simulink model "gm_comm8qamtxrxhdl"  (R2025b)
settings: Solver=FixedStepDiscrete  StartTime=0.0  StopTime=20000*qam_params.symbolPeriod  RelTol=1e-3
PreLoadFcn:
  | qam_params = comm8qamtxrxhdl_init;
InitFcn:
  | qam_params = comm8qamtxrxhdl_init;
undefined symbols (not defined in the file or in its folder): Add, Shift
libraries: simulink x4, hdlsllib x4, dspsigops x2, commchan3 x1, commrflib2 x1, dsphdlmathfun2 x1, dsphdlsigops2 x1, dspmlti4 x1, simulink_need_slupdate x1, hdlmdlgenlib x1, commdigbbndam3 x1, commsequence2 x1
(part 1 of 3)
settings Model: Creator=The MathWorks, Inc.  LastModifiedBy=Ubaid
settings SolverCC: AlgebraicLoopSolver=TrustRegion  MaxZcPerStep=1.0
settings DataIOCC: LimitDataPoints=on  SaveFormat=Array  SaveOutput=off  SaveTime=off  ReturnWorkspaceOutputs=off
settings OptimizationCC: BlockReduction=off  ConditionallyExecuteInputs=off  DefaultParameterBehavior=Inlined  ReuseModelBlockBuffer=off  LifeSpan=inf
settings DebuggingCC: AlgebraicLoopMsg=error  UnderspecifiedInitializationDetection=Classic  MergeDetectMultiDrivingBlocksExec=none  SolverPrmCheckMsg=warning  InheritedTsInSrcMsg=none  MultiTaskDSMMsg=warning  MultiTaskCondExecSysMsg=none  SingleTaskRateTransMsg=error  IntegerOverflowMsg=none  ParameterPrecisionLossMsg=none  UnconnectedInputMsg=warning  UnconnectedOutputMsg=warning  UnconnectedLineMsg=warning  AllowSymbolicDim=off  StateNameClashWarn=warning  SFUnexpectedBacktrackingDiag=warning  SFNoUnconditionalDefaultTransitionDiag=warning  SFExecutionAtInitializationDiag=none  IntegerSaturationMsg=none  ArithmeticOperatorsInVariantConditions=warning
settings HardwareCC: ProdBitPerPointer=32.0  ProdBitPerSizeT=32.0  ProdBitPerPtrDiffT=32.0  ProdLargestAtomicFloat=None  ProdIntDivRoundTo=Undefined  ProdEndianess=Unspecified  ProdWordSize=32.0  ProdHWDeviceType=ASIC/FPGA->ASIC/FPGA  ProdEqTarget=off
settings ModelReferenceCC: EnableRefExpFcnMdlSchedulingChecks=on  PropagateSignalLabelsOutOfModel=off
settings SFSimCC: SimUseLocalCustomCode=off  CustomCodeUndefinedFunction=UseInterfaceOnly
settings RTWCC: RTWUseLocalCustomCode=off  GPUComputeCapability=3.5  DLArmComputeVersion=19.05
settings CodeAppCC: StateflowObjectComments=on
settings GRTTargetCC: TargetLangStandard=C89/C90 (ANSI)
settings ConfigComp: CovMetricSettings=dw  CovSaveCumulativeToWorkspaceVar=on  CovSaveSingleToWorkspaceVar=on  CovExternalEMLEnable=off  CovSFcnEnable=off

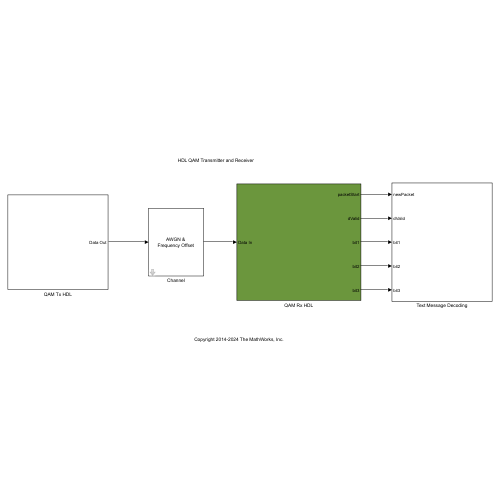
[thumbnail: Simulink's stored preview of the top-level diagram]
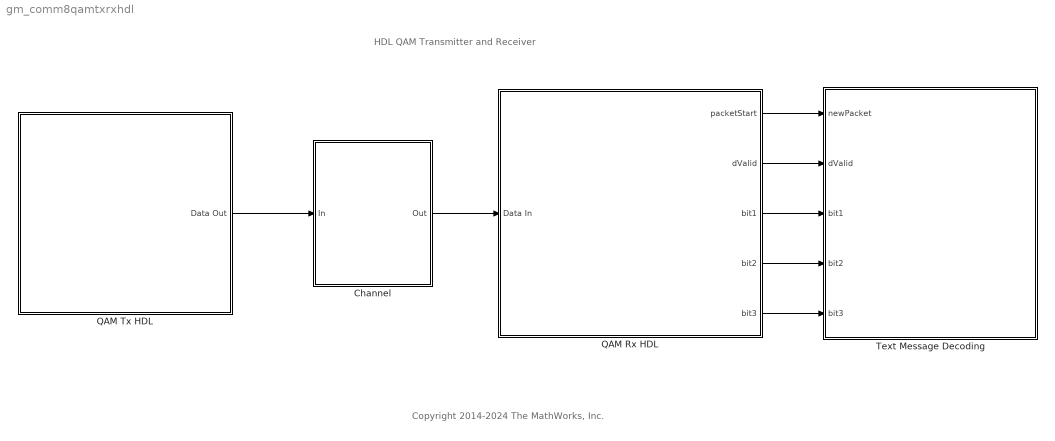
== system gm_comm8qamtxrxhdl ==
  note: HDL QAM Transmitter and Receiver
  note: Copyright 2014-2024 The MathWorks, Inc.
  Channel : Subsystem  mask{Poff=qam_params.phaseOffset, Foff=qam_params.frequencyOffset, EbNo=qam_params.EbNo, Chan_Gain=qam_params.channelGain, Chan_Delay=qam_params.channelDelay}
      mask prompts: Poff "Phase offset (deg)"; Foff "Frequency offset (Hz)"; EbNo "Eb/No"; Chan_Gain "Channel Gain"; Chan_Delay "Channel Delay"
      mask Display: disp('AWGN &\nFrequency Offset');
  QAM Rx HDL : Subsystem
  QAM Tx HDL : Subsystem
  Text Message Decoding : Subsystem
  wires:
  QAM Tx HDL/1(Data Out) -> Channel/1(In)
  Channel/1(Out) -> QAM Rx HDL/1(Data In)
  QAM Rx HDL/2(dValid) -> Text Message Decoding/2(dValid)
  QAM Rx HDL/5(bit3) -> Text Message Decoding/5(bit3)
  QAM Rx HDL/4(bit2) -> Text Message Decoding/4(bit2)
  QAM Rx HDL/3(bit1) -> Text Message Decoding/3(bit1)
  QAM Rx HDL/1(packetStart) -> Text Message Decoding/1(newPacket)

== system gm_comm8qamtxrxhdl/Channel ==
  In : Inport
  AWGN Channel2 : commchan3/AWGN Channel  LegacyMode=on  NoiseMethod="Signal to noise ratio  (Eb/No)"  noiseMode="Signal to noise ratio  (SNR)"  EbNo=EbNo  EsNo=15  SNR=15  BitsPerSymbol=3  SignalPower=0.11  SpecifySymbolPeriod=off  SamplesPerSymbol=1  SymbolPeriod=1/qam_params.sampleRate  VarianceSource=Parameter  Variance=1  RandomStream=Global stream  Seed=67  SimulateUsing=Code generation
  Constant : Constant  Value=Chan_Delay  SampleTime=1/qam_params.sampleRate
  Data Type Conversion1 : DataTypeConversion  OutDataTypeStr=fixdt(1,16,15)  SaturateOnIntegerOverflow=off  RndMeth=Floor
  Data Type Conversion4 : DataTypeConversion  OutDataTypeStr=double  SaturateOnIntegerOverflow=off  RndMeth=Floor
  Gain : Gain  Gain=Chan_Gain
  Phase/ Frequency Offset1 : commrflib2/Phase// Frequency Offset  phaseOffset=Poff  freqPort=off  freqOffset=Foff
  Variable Fractional Delay : dspsigops/Variable Fractional Delay  mode=OBSOLETE  modeActive=Linear  L=4  FarrowL=4  R=10  alpha=1  dmax=56*4  ic=0  noDFT=off  fallbackFIR=Clip to the minimum value necessary for centered kernel  fallbackFarrow=Clip to the minimum value necessary for centered kernel  roundingMode=Zero  overflowMode=off
  Out : Outport  VectorParamsAs1DForOutWhenUnconnected=off
  wires:
  Gain/1 -> Data Type Conversion1/1
  Constant/1 -> Variable Fractional Delay/2
  Variable Fractional Delay/1 -> AWGN Channel2/1
  Phase/ Frequency Offset1/1 -> Variable Fractional Delay/1
  Data Type Conversion4/1 -> Phase/ Frequency Offset1/1
  Data Type Conversion1/1 -> Out/1
  AWGN Channel2/1 -> Gain/1
  In/1 -> Data Type Conversion4/1

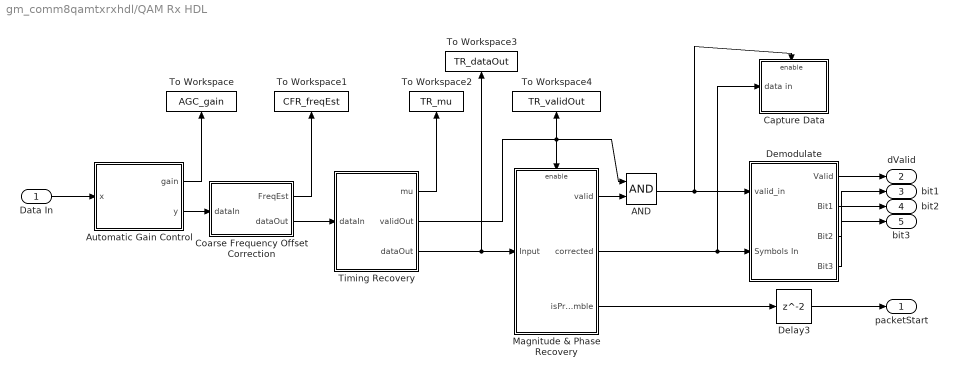
== system gm_comm8qamtxrxhdl/QAM Rx HDL ==
  Data In : Inport
  AND : Logic  AllPortsSameDT=off  OutDataTypeStr=boolean
  Automatic Gain Control : Subsystem  mask{AGC_Ref=.23, AGC_Gain=0.001}
      mask prompts: AGC_Ref "Target Amplitude"; AGC_Gain "AGC Loop Gain"
  Capture Data : Subsystem
  Coarse Frequency Offset Correction : Subsystem
  Delay3 : Delay  InitialCondition=0
  Demodulate : Subsystem
  Magnitude & Phase Recovery : Subsystem  mask{PreAmb=qam_params.preambleRx.', threshold=1.1, LMS_Step=1/4}
      mask prompts: PreAmb "Preamble symbols"; LMS_Step "LMS step size"
  Timing Recovery : Subsystem
  To Workspace : ToWorkspace  VariableName=AGC_gain  SaveFormat=Timeseries  SampleTime=-1
  To Workspace1 : ToWorkspace  VariableName=CFR_freqEst  SaveFormat=Timeseries  SampleTime=-1
  To Workspace2 : ToWorkspace  VariableName=TR_mu  SaveFormat=Timeseries  SampleTime=-1
  To Workspace3 : ToWorkspace  VariableName=TR_dataOut  SaveFormat=Timeseries  SampleTime=-1
  To Workspace4 : ToWorkspace  VariableName=TR_validOut  SaveFormat=Timeseries  SampleTime=-1
  packetStart : Outport  VectorParamsAs1DForOutWhenUnconnected=off
  dValid : Outport  Port=2  VectorParamsAs1DForOutWhenUnconnected=off
  bit1 : Outport  Port=3  VectorParamsAs1DForOutWhenUnconnected=off
  bit2 : Outport  Port=4  VectorParamsAs1DForOutWhenUnconnected=off
  bit3 : Outport  Port=5  VectorParamsAs1DForOutWhenUnconnected=off
  wires:
  Timing Recovery/1(mu) -> To Workspace2/1
  Coarse Frequency Offset Correction/1(FreqEst) -> To Workspace1/1
  Magnitude & Phase Recovery/2(corrected) -> Capture Data/1(data in), Demodulate/2(Symbols In)
  AND/1 -> Capture Data/Enable, Demodulate/1(valid_in)
  Magnitude & Phase Recovery/1(valid) -> AND/2
  Delay3/1 -> packetStart/1
  Coarse Frequency Offset Correction/2(dataOut) -> Timing Recovery/1(dataIn)
  Automatic Gain Control/2(y) -> Coarse Frequency Offset Correction/1(dataIn)
  Automatic Gain Control/1(gain) -> To Workspace/1
  Data In/1 -> Automatic Gain Control/1(x)
  Timing Recovery/2(validOut) -> Magnitude & Phase Recovery/Enable, To Workspace4/1, AND/1
  Demodulate/1(Valid) -> dValid/1
  Magnitude & Phase Recovery/3(isPreamble) -> Delay3/1
  Demodulate/4(Bit3) -> bit3/1
  Demodulate/3(Bit2) -> bit2/1
  Demodulate/2(Bit1) -> bit1/1
  Timing Recovery/3(dataOut) -> To Workspace3/1, Magnitude & Phase Recovery/1(Input)

== system gm_comm8qamtxrxhdl/QAM Tx HDL ==
  " Zero" : Constant  Value="fi(0,1,16,15,\"hex\",\"0000 + 0000 i\")"  OutDataTypeStr=fixdt(1, 16, 15)  SampleTime=1e-06
  Data Generation & Packetization : Subsystem
  Input Mux : MultiPortSwitch  DataPortOrder=Zero-based contiguous  Inputs=2  DiagnosticForDefault=None  zeroidx=on  OutDataTypeStr=fixdt(1, 16, 15)  SampleTime=1e-06  SaturateOnIntegerOverflow=off  InputSameDT=off
  Pipeline{1..4} (4 alike) : Delay  DelayLength=double(1)  InitialCondition=0  SampleTime=1e-06
  Pipeline5 : RateTransition  InitialCondition=double(0)  OutPortSampleTimeOpt=Multiple of input port sample time  OutPortSampleTimeMultiple=3
  Pipeline5_absorbed : Delay  DelayLength=0
  Pulse Shaping : Subsystem
  Symbol Mapping : Subsystem
  crp_out_delay : Delay  DelayLength=double(1)  InitialCondition=0  SampleTime=8.33333333333333e-08
  Data Out : Outport  SampleTime=2.5e-07  VectorParamsAs1DForOutWhenUnconnected=off
  wires:
  Data Generation & Packetization/1(Valid Out) -> Pipeline1/1
  Data Generation & Packetization/2(Raw Data) -> Pipeline2/1
  Symbol Mapping/1(Valid out) -> Pipeline3/1
  Pipeline1/1 -> Symbol Mapping/1(Valid In)
  Symbol Mapping/2(Symbol Out) -> Pipeline4/1
  Pipeline2/1 -> Symbol Mapping/2(Integer In)
  Pipeline3/1 -> Input Mux/1
  " Zero"/1 -> Input Mux/2
  Pipeline4/1 -> Input Mux/3
  Input Mux/1 -> Pulse Shaping/1(dataIn)
  Pulse Shaping/1(dataOut) -> crp_out_delay/1
  crp_out_delay/1 -> Pipeline5/1
  Pipeline5/1 -> Pipeline5_absorbed/1
  Pipeline5_absorbed/1 -> Data Out/1

== system gm_comm8qamtxrxhdl/Text Message Decoding ==
  newPacket : Inport
  dValid : Inport  Port=2
  bit1 : Inport  Port=3
  bit2 : Inport  Port=4
  bit3 : Inport  Port=5
  " " : MATLAB Function  TreatAsAtomicUnit=on
  Descramble and Print : Subsystem  TreatAsAtomicUnit=on
  wires:
  newPacket/1 -> " "/1(newPacket)
  dValid/1 -> " "/2(dValid)
  bit3/1 -> " "/5(bit3)
  " "/1(RxGo) -> Descramble and Print/Enable
  " "/2(framed_data) -> Descramble and Print/1(In1)
  bit2/1 -> " "/4(bit2)
  bit1/1 -> " "/3(bit1)

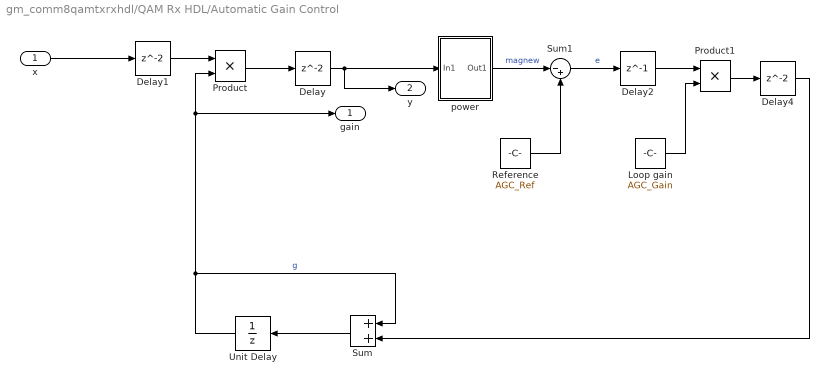
== system gm_comm8qamtxrxhdl/QAM Rx HDL/Automatic Gain Control ==
  x : Inport
  Delay : Delay  InitialCondition=0
  Delay1 : Delay  InitialCondition=0
  Delay2 : Delay  DelayLength=1  InitialCondition=0
  Delay4 : Delay  InitialCondition=0
  Loop gain : Constant  Value=AGC_Gain  OutDataTypeStr=fixdt(1,16,15)  SampleTime=1/qam_params.sampleRate
  Product : Product  OutDataTypeStr=fixdt(1,16,15)  SaturateOnIntegerOverflow=on
  Product1 : Product  OutDataTypeStr=fixdt(1,16,15)  SaturateOnIntegerOverflow=on
  Reference : Constant  Value=AGC_Ref  OutDataTypeStr=fixdt(1,16,15)  SampleTime=1/qam_params.sampleRate
  Sum : Sum  OutDataTypeStr=Inherit: Same as accumulator  AccumDataTypeStr=fixdt(1,24,15)  SaturateOnIntegerOverflow=on
  Sum1 : Sum  Inputs=|-+  OutDataTypeStr=Inherit: Same as first input
  Unit Delay : UnitDelay  InitialCondition=.5  SampleTime=-1  HasFrameUpgradeWarning=on
  power : Subsystem
  gain : Outport  VectorParamsAs1DForOutWhenUnconnected=off
  y : Outport  Port=2  PortDimensions=1  VectorParamsAs1DForOutWhenUnconnected=off
  wires:
  Delay1/1 -> Product/1
  power/1(Out1) -> Sum1/1  "magnew"
  Reference/1 -> Sum1/2
  Sum/1 -> Unit Delay/1
  Loop gain/1 -> Product1/2
  x/1 -> Delay1/1
  Delay4/1 -> Sum/2
  Unit Delay/1 -> Sum/1, Product/2, gain/1  "g"
  Product1/1 -> Delay4/1
  Delay2/1 -> Product1/1
  Sum1/1 -> Delay2/1  "e"
  Delay/1 -> power/1(In1), y/1
  Product/1 -> Delay/1

== system gm_comm8qamtxrxhdl/QAM Rx HDL/Capture Data ==
  data in : Inport
  Enable : EnablePort
  To Workspace2 : ToWorkspace  VariableName=symbolEstimates  SaveFormat=Timeseries  SampleTime=-1
  wires:
  data in/1 -> To Workspace2/1

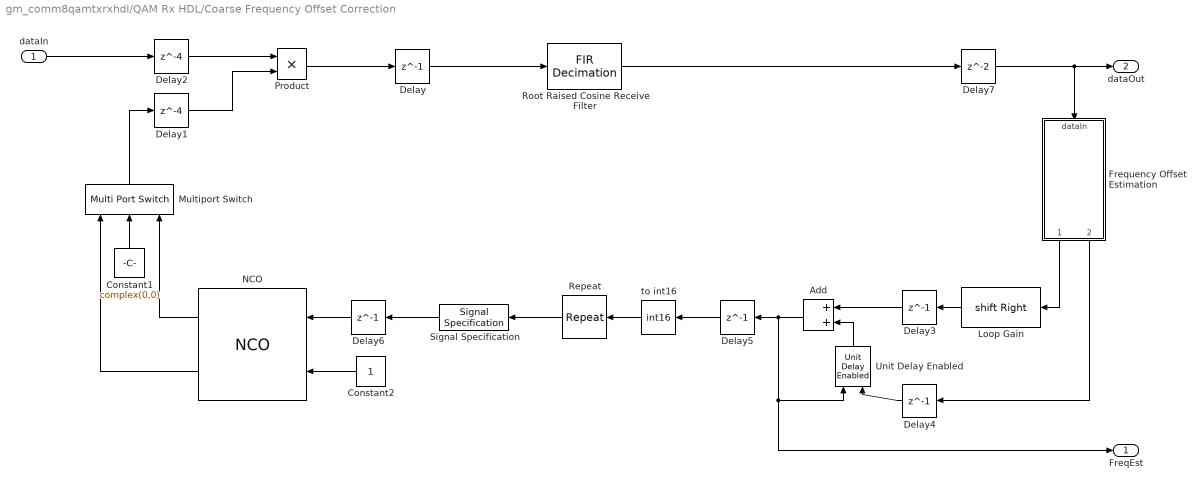
== system gm_comm8qamtxrxhdl/QAM Rx HDL/Coarse Frequency Offset Correction ==
  dataIn : Inport
  Add : Sum  AccumDataTypeStr=fixdt(1,16,3)
  Constant1 : Constant  Value=complex(0,0)  OutDataTypeStr=fixdt(1,16,15)  SampleTime=1/qam_params.sampleRate
  Constant2 : Constant  OutDataTypeStr=boolean  SampleTime=1/qam_params.sampleRate
  Delay{,3..6} (5 alike) : Delay  DelayLength=1  InitialCondition=0
  Delay1 : Delay  DelayLength=4  InitialCondition=0
  Delay2 : Delay  DelayLength=4  InitialCondition=0
  Delay7 : Delay  InitialCondition=0
  Frequency Offset Estimation : Subsystem  mask{M=64, N=256, avFilterCoeffs=0}
      mask prompts: M "M (Luise Parameter)"; N "N (Luise Parameter)"; avFilterCoeffs "Filter Coeffs"
      mask init:
      | avFilterCoeffs = 1./(N*ones(1,M));
  Loop Gain : ArithShift  BinPtShiftNumber=-3  BitShiftDirection=Right
  Multiport Switch : MultiPortSwitch  DataPortOrder=Zero-based contiguous  Inputs=2  zeroidx=on  SaturateOnIntegerOverflow=off  InputSameDT=off
  NCO : dsphdlsigops2/NCO  PhaseIncrementSource=Input port  PhaseIncrement=100  PhaseOffsetSource=Property  PhaseOffset=0  DitherSource=Property  NumDitherBits=4  SamplesPerFrame=1  LUTCompress=off  ResetAction=off  Waveform=Complex exponential  PhasePort=off  SimulateUsing=Code generation  AccumulatorWL=16  PhaseQuantization=on  NumQuantizerAccumulatorBits=16  OutputDataType=Binary point scaling  OutputWL=16  OutputFL=15
  Product : Product  OutDataTypeStr=fixdt(1,16,15)
  Repeat : dspsigops/Repeat  FactorSource=Dialog parameter  N=2  Nmax=16  InputProcessing=Columns as channels (frame based)  RateOptions=Allow multirate processing  ic=0  mode=Unused parameter value
  Root Raised Cosine Receive Filter : dspmlti4/FIR Decimation  FilterSource=Dialog parameters  h=qam_params.ReceiverFilterCoefficients  D=2  filtStruct=Direct form transposed  FilterObject=Hm_firdecim  framing=Allow multirate processing  AllowArbitraryInputLength=off  inputOffset=0  outputBufInitCond=0  roundingMode=Floor  overflowMode=off  firstCoeffDataTypeStr=Inherit: Same word length as input  firstCoeffMin=[]  firstCoeffMax=[]  firstCoeffLastDataTypeStr=Inherit: Same word length as input  prodOutputMode=Binary point scaling  prodOutputWordLength=16  prodOutputFracLength=15  prodOutputDataTypeStr=fixdt(1,16,15)  prodOutputLastDataTypeStr=fixdt(1,16,15)  accumMode=Binary point scaling  accumWordLength=16  accumFracLength=15  accumDataTypeStr=fixdt(1,16,15)  accumLastDataTypeStr=fixdt(1,16,15)  outputMode=Binary point scaling  outputWordLength=16  outputFracLength=15  outputDataTypeStr=fixdt(1,16,15)  outputMin=[]  outputMax=[]  outputLastDataTypeStr=fixdt(1,16,15)
  Signal Specification : SignalSpecification  OutDataTypeStr=int16  Dimensions=1
  Unit Delay Enabled : simulink_need_slupdate/Unit Delay Enabled  vinit=0.0  tsamp=-1
  to int16 : DataTypeConversion  OutDataTypeStr=int16  SaturateOnIntegerOverflow=off  RndMeth=Floor
  FreqEst : Outport  VectorParamsAs1DForOutWhenUnconnected=off
  dataOut : Outport  Port=2  VectorParamsAs1DForOutWhenUnconnected=off
  wires:
  Delay5/1 -> to int16/1
  Constant1/1 -> Multiport Switch/2
  Multiport Switch/1 -> Delay1/1
  NCO/2 -> Multiport Switch/1
  NCO/1 -> Multiport Switch/3
  Delay6/1 -> NCO/1
  Delay7/1 -> Frequency Offset Estimation/1(dataIn), dataOut/1
  Unit Delay Enabled/1 -> Add/2
  Delay4/1 -> Unit Delay Enabled/2
  Delay3/1 -> Add/1
  Delay2/1 -> Product/1
  Delay1/1 -> Product/2
  Delay/1 -> Root Raised Cosine Receive Filter/1
  Add/1 -> Delay5/1, Unit Delay Enabled/1, FreqEst/1
  to int16/1 -> Repeat/1
  Repeat/1 -> Signal Specification/1
  Frequency Offset Estimation/1(Estimate) -> Loop Gain/1
  Signal Specification/1 -> Delay6/1
  Constant2/1 -> NCO/2
  Frequency Offset Estimation/2(Estimate Valid) -> Delay4/1
  Loop Gain/1 -> Delay3/1
  Root Raised Cosine Receive Filter/1 -> Delay7/1
  dataIn/1 -> Delay2/1
  Product/1 -> Delay/1

== system gm_comm8qamtxrxhdl/QAM Rx HDL/Demodulate ==
  valid_in : Inport
  Symbols In : Inport  Port=2
  Delay{1..4} (4 alike) : Delay  DelayLength=1  InitialCondition=0
  Demux : Demux  Outputs=3
  Rectangular QAM Demodulator Baseband : MATLAB Function  TreatAsAtomicUnit=on
  Shift Arithmetic : ArithShift  BinPtShiftNumber=2  BitShiftDirection=Right
  Valid : Outport  VectorParamsAs1DForOutWhenUnconnected=off
  Bit1 : Outport  Port=2  VectorParamsAs1DForOutWhenUnconnected=off
  Bit2 : Outport  Port=3  VectorParamsAs1DForOutWhenUnconnected=off
  Bit3 : Outport  Port=4  VectorParamsAs1DForOutWhenUnconnected=off
  wires:
  Rectangular QAM Demodulator Baseband/1(y) -> Delay1/1
  Delay4/1 -> Rectangular QAM Demodulator Baseband/1(u)
  Delay3/1 -> Delay2/1
  Delay2/1 -> Valid/1
  Delay1/1 -> Demux/1
  Shift Arithmetic/1 -> Delay4/1
  Symbols In/1 -> Shift Arithmetic/1
  Demux/3 -> Bit3/1
  Demux/2 -> Bit2/1
  valid_in/1 -> Delay3/1
  Demux/1 -> Bit1/1

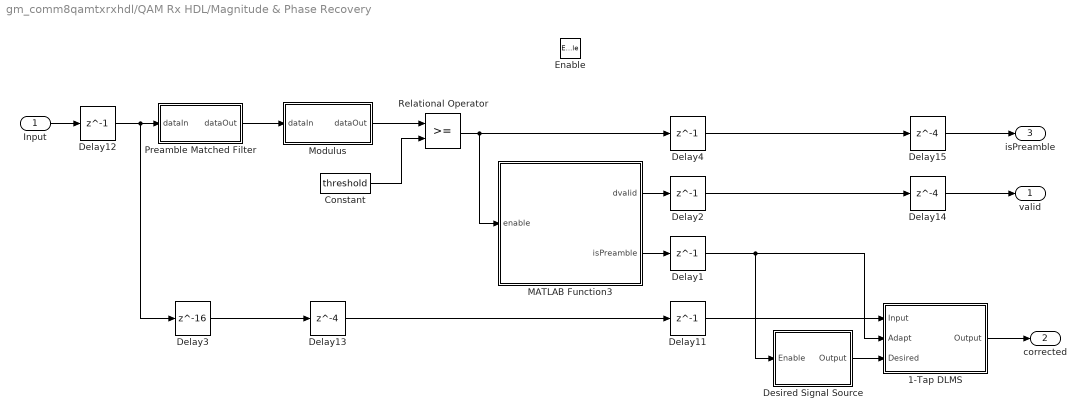
== system gm_comm8qamtxrxhdl/QAM Rx HDL/Magnitude & Phase Recovery ==
  Input : Inport
  Enable : EnablePort
  1-Tap DLMS : Subsystem
  Constant : Constant  Value=threshold  OutDataTypeStr=Inherit: Inherit via back propagation  SampleTime=1/(qam_params.sampleRate/2)
  Delay{1..2,4,11..12} (5 alike) : Delay  DelayLength=1  InitialCondition=0
  Delay13 : Delay  DelayLength=4  InitialCondition=0
  Delay14 : Delay  DelayLength=4  InitialCondition=0
  Delay15 : Delay  DelayLength=4  InitialCondition=0
  Delay3 : Delay  DelayLength=16  InitialCondition=0
  Desired Signal Source : Subsystem
  MATLAB Function3 : MATLAB Function  TreatAsAtomicUnit=on
  Modulus : Subsystem
  Preamble Matched Filter : Subsystem
  Relational Operator : RelationalOperator  OutDataTypeStr=boolean
  valid : Outport  InitialOutput=0  VectorParamsAs1DForOutWhenUnconnected=off
  corrected : Outport  Port=2  InitialOutput=0  VectorParamsAs1DForOutWhenUnconnected=off
  isPreamble : Outport  Port=3  InitialOutput=0  VectorParamsAs1DForOutWhenUnconnected=off
  wires:
  Desired Signal Source/1(Output) -> 1-Tap DLMS/3(Desired)
  Delay1/1 -> Desired Signal Source/1(Enable), 1-Tap DLMS/2(Adapt)
  1-Tap DLMS/1(Output) -> corrected/1
  Delay13/1 -> Delay11/1
  Delay11/1 -> 1-Tap DLMS/1(Input)
  Delay12/1 -> Preamble Matched Filter/1(dataIn), Delay3/1
  Delay4/1 -> Delay15/1
  Delay2/1 -> Delay14/1
  Delay15/1 -> isPreamble/1
  Delay14/1 -> valid/1
  Delay3/1 -> Delay13/1
  Input/1 -> Delay12/1
  Preamble Matched Filter/1(dataOut) -> Modulus/1(dataIn)
  Constant/1 -> Relational Operator/2
  Relational Operator/1 -> Delay4/1, MATLAB Function3/1(enable)
  Modulus/1(dataOut) -> Relational Operator/1
  MATLAB Function3/2(isPreamble) -> Delay1/1
  MATLAB Function3/1(dvalid) -> Delay2/1

== system gm_comm8qamtxrxhdl/QAM Rx HDL/Timing Recovery ==
  dataIn : Inport
  Delay1 : Delay  DelayLength=1
  Delay2 : Delay  DelayLength=1
  Delay5 : Delay  DelayLength=6
  Gain : Gain  Gain=-2^-8  OutDataTypeStr=fixdt(1,16,15)
  Integer Delay3 : Delay  DelayLength=1
  Integer Delay4 : Delay  DelayLength=1
  Interpolation Control : MATLAB Function
  "Interpolation Filter " : Subsystem
  Timing Error Detector : MATLAB Function  TreatAsAtomicUnit=on
  mu : Outport  VectorParamsAs1DForOutWhenUnconnected=off
  validOut : Outport  Port=2  VectorParamsAs1DForOutWhenUnconnected=off
  dataOut : Outport  Port=3  VectorParamsAs1DForOutWhenUnconnected=off
  wires:
  Delay2/1 -> Gain/1
  Delay1/1 -> Interpolation Control/1(Delta)
  Delay5/1 -> "Interpolation Filter "/1(dataIn)
  dataIn/1 -> Delay5/1
  "Interpolation Filter "/1(dataOut) -> dataOut/1, Timing Error Detector/1(In)
  Timing Error Detector/1(e) -> Delay2/1
  Gain/1 -> Delay1/1
  Integer Delay4/1 -> "Interpolation Filter "/2(mu), mu/1
  "Interpolation Filter "/2(validOut) -> validOut/1, Timing Error Detector/2(strobe)
  Integer Delay3/1 -> "Interpolation Filter "/3(validIn)
  Interpolation Control/1(Underflow) -> Integer Delay3/1
  Interpolation Control/2(mu) -> Integer Delay4/1

== system gm_comm8qamtxrxhdl/QAM Tx HDL/Data Generation & Packetization ==
  Controller FSM : Subsystem
  Data Source : Subsystem
  Downsample : DownSample  N=double(3)  phase=double(0)  RateOptions=Allow multirate processing  AllowArbitraryFixedInput=on
  Group Bits : Subsystem
  Pipeline : Delay  DelayLength=double(2)  InitialCondition=0  SampleTime=3.33333333333333e-07
  Pipeline1 : Delay  DelayLength=double(1)  InitialCondition=0  SampleTime=3.33333333333333e-07
  Pipeline2 : Delay  DelayLength=double(1)  InitialCondition=0  SampleTime=3.33333333333333e-07
  Valid : Constant  OutDataTypeStr=boolean  SampleTime=3.33333333333333e-07
  Valid Out : Outport  SampleTime=1e-06  VectorParamsAs1DForOutWhenUnconnected=off
  Raw Data : Outport  Port=2  SampleTime=1e-06  VectorParamsAs1DForOutWhenUnconnected=off
  wires:
  Controller FSM/1(reset_preamble) -> Data Source/1(reset preamble)
  Valid/1 -> Pipeline/1
  Controller FSM/2(load_preamble) -> Data Source/2(load preamble)
  Controller FSM/3(load_data) -> Data Source/3(load data)
  Data Source/1(packet_bits) -> Pipeline2/1
  Pipeline/1 -> Pipeline1/1
  Pipeline1/1 -> Downsample/1
  Pipeline2/1 -> Group Bits/1(Bits In)
  Downsample/1 -> Valid Out/1
  Group Bits/1(Integer Out) -> Raw Data/1

== system gm_comm8qamtxrxhdl/QAM Tx HDL/Pulse Shaping ==
  dataIn : Inport  OutDataTypeStr=fixdt(1, 16, 15)  PortDimensions=1  SampleTime=1e-06
      settings: SignalType=complex
  RRC Interpolation Filter : Subsystem
  dataOut : Outport  SampleTime=8.33333333333333e-08  VectorParamsAs1DForOutWhenUnconnected=off
  wires:
  dataIn/1 -> RRC Interpolation Filter/1(RRC Interpolation Filter_In)
  RRC Interpolation Filter/1(RRC Interpolation Filter_out) -> dataOut/1

== system gm_comm8qamtxrxhdl/QAM Tx HDL/Symbol Mapping ==
  Valid In : Inport  OutDataTypeStr=boolean  PortDimensions=1  SampleTime=1e-06
  Integer In : Inport  Port=2  OutDataTypeStr=fixdt(0, 3, 0)  PortDimensions=1  SampleTime=1e-06
  Rectangular QAM Modulator Baseband : commdigbbndam3/Rectangular QAM Modulator Baseband  M=8  InType=Integer  Enc=Gray  Mapping=[0:15]  PowType=Min. distance between symbols  MinDist=0.5  AvgPow=.66  PeakPow=1.1  Ph=0  outDtype=Fixed-point  outWordLen=16  outUDDataType=sfix(16)  outFracLenMode=Best precision  outFracLen=15  outDataTypeStr=fixdt(1,16)  outLastDataTypeStr=fixdt(1,16)
  Valid out : Outport  SampleTime=1e-06  VectorParamsAs1DForOutWhenUnconnected=off
  Symbol Out : Outport  Port=2  SampleTime=1e-06  VectorParamsAs1DForOutWhenUnconnected=off
  wires:
  Integer In/1 -> Rectangular QAM Modulator Baseband/1
  Valid In/1 -> Valid out/1
  Rectangular QAM Modulator Baseband/1 -> Symbol Out/1

== system gm_comm8qamtxrxhdl/Text Message Decoding/Descramble and Print ==
  In1 : Inport
  Enable : EnablePort
  BitsToDecimal1 : MATLAB Function  TreatAsAtomicUnit=on
  Descrambler : commsequence2/Descrambler  M=2  poly=[1 1 1 0 1]  iniStaSource=Dialog Parameter  ini_sta=[0 0 0 0]  resetViaPort=off
  Selector : Selector  IndexOptions=Index vector (dialog)  Indices=[43:1:168]  OutputSizes=1
  Selector1 : Selector  IndexOptions=Index vector (dialog)  Indices=[1:1:126]  OutputSizes=1
  wires:
  Descrambler/1 -> Selector1/1
  Selector/1 -> Descrambler/1
  In1/1 -> Selector/1
  Selector1/1 -> BitsToDecimal1/1(u)

== system gm_comm8qamtxrxhdl/QAM Rx HDL/Automatic Gain Control/power ==
  In1 : Inport
  Complex to Real-Imag : ComplexToRealImag
  Delay : Delay  InitialCondition=0
  Delay1 : Delay  InitialCondition=0
  Delay2 : Delay  InitialCondition=0
  Product3 : Product  OutDataTypeStr=fixdt(1,16,15)  SaturateOnIntegerOverflow=on
  Product4 : Product  OutDataTypeStr=fixdt(1,16,15)  SaturateOnIntegerOverflow=on
  Sum1 : Sum  OutDataTypeStr=fixdt(1,16,14)  AccumDataTypeStr=fixdt(1,16,15)  SaturateOnIntegerOverflow=on
  Out1 : Outport  VectorParamsAs1DForOutWhenUnconnected=off
  wires:
  Delay2/1 -> Out1/1
  In1/1 -> Complex to Real-Imag/1
  Delay1/1 -> Sum1/2
  Delay/1 -> Sum1/1
  Sum1/1 -> Delay2/1
  Product4/1 -> Delay1/1
  Complex to Real-Imag/2 -> Product4/2, Product4/1
  Complex to Real-Imag/1 -> Product3/1, Product3/2
  Product3/1 -> Delay/1

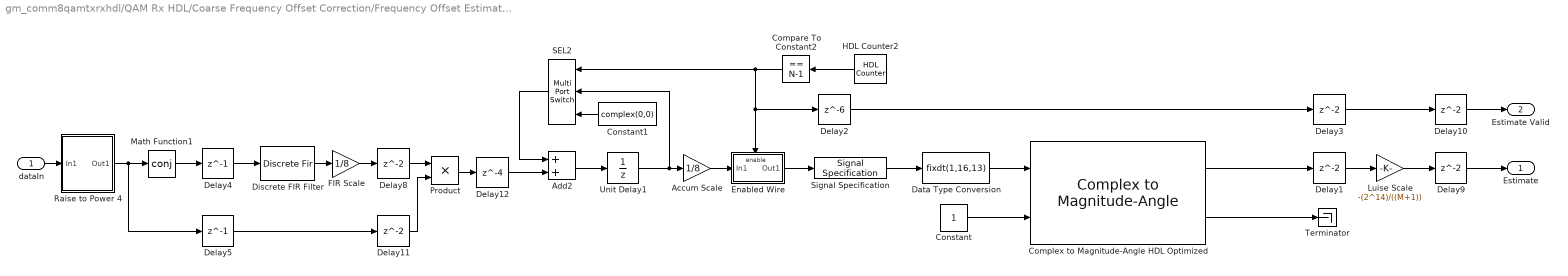
== system gm_comm8qamtxrxhdl/QAM Rx HDL/Coarse Frequency Offset Correction/Frequency Offset Estimation ==
  dataIn : Inport
  Accum Scale : Gain  Gain=1/8  OutDataTypeStr=fixdt(1,32,31)
  Add2 : Sum  OutDataTypeStr=fixdt(1,32,28)
  Compare To Constant2 : simulink/Logic and Bit Operations/Compare To Constant  relop===  const=N-1  OutDataTypeStr=boolean
  Complex to Magnitude-Angle HDL Optimized : dsphdlmathfun2/Complex to Magnitude-Angle  NumIterationsSource=Property  NumIterations=5  OutputFormat=Angle  AngleFormat=Normalized  ScaleOutput=on  ScalingMethod=Shift-Add  SimulateUsing=Code generation
  Constant : Constant  OutDataTypeStr=boolean  SampleTime=5e-7
  Constant1 : Constant  Value=complex(0,0)  OutDataTypeStr=fixdt(1,32,28)  SampleTime=1/(qam_params.sampleRate/2)
  Data Type Conversion : DataTypeConversion  OutDataTypeStr=fixdt(1,16,13)  SaturateOnIntegerOverflow=off  RndMeth=Floor
  Delay{1,3,8..11} (6 alike) : Delay  InitialCondition=0
  Delay12 : Delay  DelayLength=4  InitialCondition=0
  Delay2 : Delay  DelayLength=6  InitialCondition=0
  Delay4 : Delay  DelayLength=1  InitialCondition=0
  Delay5 : Delay  DelayLength=1  InitialCondition=0
  Discrete FIR Filter : DiscreteFir  FilterStructure=Direct form transposed  Coefficients=ones(1,M)  CoefDataTypeStr=fixdt(1,2,0)  ProductDataTypeStr=fixdt(1,16,15)  AccumDataTypeStr=fixdt(1,19,15)  OutDataTypeStr=fixdt(1,19,15)
  Enabled Wire : Subsystem  TreatAsAtomicUnit=on
  FIR Scale : Gain  Gain=1/8  OutDataTypeStr=fixdt(1,19,18)
  HDL Counter2 : hdlsllib/Sources/HDL Counter  CountType=Count limited  CountInit=0  CountStep=1  CountMax=N-1  CountFromType=Initial value  CountFrom=0  CountResetPort=off  CountLoadPort=off  CountEnbPort=off  CountDirPort=off  CountHitOutputPort=off  CountDataType=Unsigned  CountWordLen=12  CountFracLen=0  CountSampTime=1/(qam_params.sampleRate/2)
  Luise Scale : Gain  Gain=-(2^14)/((M+1))  OutDataTypeStr=int16
  Math Function1 : Math  Operator=conj  SignedPower=on  OutputSignalType=complex
  Product : Product  OutDataTypeStr=fixdt(1,32,31)
  Raise to Power 4 : Subsystem
  SEL2 : MultiPortSwitch  DataPortOrder=Zero-based contiguous  Inputs=2  DiagnosticForDefault=None  zeroidx=on  OutDataTypeStr=fixdt(1,32,28)  SaturateOnIntegerOverflow=off  InputSameDT=off
  Signal Specification : SignalSpecification  Dimensions=1
  Terminator : Terminator
  Unit Delay1 : UnitDelay  InitialCondition=0+0j  SampleTime=-1  HasFrameUpgradeWarning=on
  Estimate : Outport  VectorParamsAs1DForOutWhenUnconnected=off
  Estimate Valid : Outport  Port=2  VectorParamsAs1DForOutWhenUnconnected=off
  wires:
  Data Type Conversion/1 -> Complex to Magnitude-Angle HDL Optimized/1
  Signal Specification/1 -> Data Type Conversion/1
  Complex to Magnitude-Angle HDL Optimized/2 -> Terminator/1
  Constant/1 -> Complex to Magnitude-Angle HDL Optimized/2
  Delay1/1 -> Luise Scale/1
  Accum Scale/1 -> Enabled Wire/1(In1)
  Compare To Constant2/1 -> Delay2/1, Enabled Wire/Enable, SEL2/1
  Delay12/1 -> Add2/2
  SEL2/1 -> Add2/1
  Unit Delay1/1 -> Accum Scale/1, SEL2/2
  Add2/1 -> Unit Delay1/1
  Constant1/1 -> SEL2/3
  Product/1 -> Delay12/1
  Delay8/1 -> Product/1
  FIR Scale/1 -> Delay8/1
  Delay5/1 -> Delay11/1
  Delay4/1 -> Discrete FIR Filter/1
  Delay11/1 -> Product/2
  Discrete FIR Filter/1 -> FIR Scale/1
  Raise to Power 4/1(Out1) -> Delay5/1, Math Function1/1
  HDL Counter2/1 -> Compare To Constant2/1
  Enabled Wire/1(Out1) -> Signal Specification/1
  Luise Scale/1 -> Delay9/1
  Math Function1/1 -> Delay4/1
  Complex to Magnitude-Angle HDL Optimized/1 -> Delay1/1
  Delay3/1 -> Delay10/1
  Delay2/1 -> Delay3/1
  dataIn/1 -> Raise to Power 4/1(In1)
  Delay10/1 -> Estimate Valid/1
  Delay9/1 -> Estimate/1

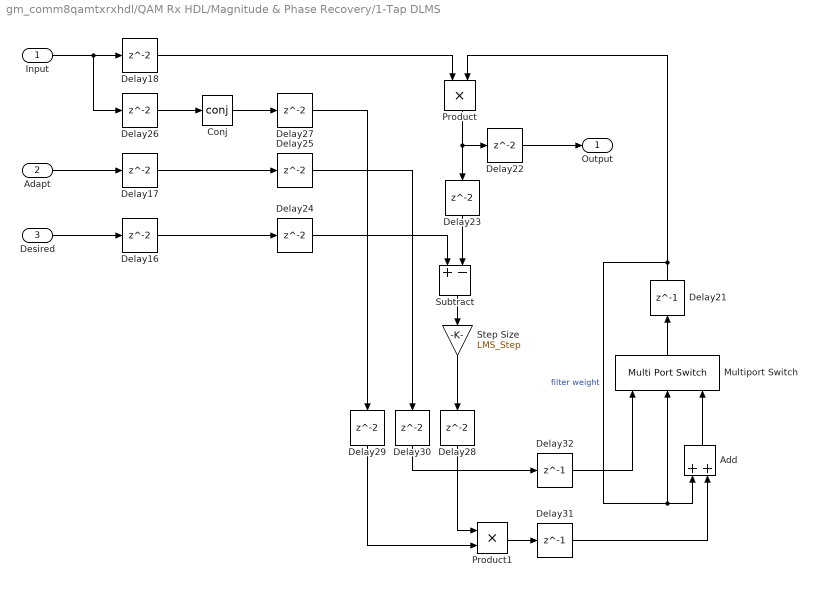
== system gm_comm8qamtxrxhdl/QAM Rx HDL/Magnitude & Phase Recovery/1-Tap DLMS ==
  Input : Inport
  Adapt : Inport  Port=2
  Desired : Inport  Port=3
  Add : Sum  OutDataTypeStr=fixdt(1,17,14)
  Conj : Math  Operator=conj  SignedPower=on
  Delay{16..18,22..30} (12 alike) : Delay  InitialCondition=0
  Delay21 : Delay  DelayLength=1  InitialCondition=1
  Delay31 : Delay  DelayLength=1  InitialCondition=0
  Delay32 : Delay  DelayLength=1  InitialCondition=0
  Multiport Switch : MultiPortSwitch  DataPortOrder=Zero-based contiguous  Inputs=2  zeroidx=on  SaturateOnIntegerOverflow=off  InputSameDT=off
  Product : Product  OutDataTypeStr=fixdt(1,16,14)
  Product1 : Product  OutDataTypeStr=fixdt(1,16,15)
  Step Size : Gain  Gain=LMS_Step  OutDataTypeStr=fixdt(1,16,15)
  Subtract : Sum  Inputs=+-  AccumDataTypeStr=fixdt(1,16,14)
  Output : Outport  VectorParamsAs1DForOutWhenUnconnected=off
  wires:
  Conj/1 -> Delay27/1
  Delay32/1 -> Multiport Switch/1
  Delay31/1 -> Add/2
  Delay30/1 -> Delay32/1
  Delay29/1 -> Product1/2
  Delay28/1 -> Product1/1
  Delay25/1 -> Delay30/1
  Delay27/1 -> Delay29/1
  Step Size/1 -> Delay28/1
  Product1/1 -> Delay31/1
  Delay22/1 -> Output/1
  Delay26/1 -> Conj/1
  Delay24/1 -> Subtract/1
  Delay23/1 -> Subtract/2
  Input/1 -> Delay18/1, Delay26/1
  Multiport Switch/1 -> Delay21/1
  Subtract/1 -> Step Size/1
  Product/1 -> Delay22/1, Delay23/1
  Delay21/1 -> Add/1, Multiport Switch/2, Product/2  "filter weight"
  Add/1 -> Multiport Switch/3
  Delay17/1 -> Delay25/1
  Delay16/1 -> Delay24/1
  Delay18/1 -> Product/1
  Desired/1 -> Delay16/1
  Adapt/1 -> Delay17/1

== system gm_comm8qamtxrxhdl/QAM Rx HDL/Magnitude & Phase Recovery/Desired Signal Source ==
  Enable : Inport
  HDL Counter2 : hdlsllib/Sources/HDL Counter  CountType=Count limited  CountInit=0  CountStep=1  CountMax=13  CountFromType=Initial value  CountFrom=0  CountResetPort=off  CountLoadPort=off  CountEnbPort=on  CountDirPort=off  CountHitOutputPort=off  CountDataType=Unsigned  CountWordLen=8  CountFracLen=0  CountSampTime=-1
  data lookup : LookupNDDirect  NumberOfTableDimensions=1  Table=PreAmb  DiagnosticForOutOfRangeInput=Error  TableDataTypeStr=fixdt(1,16,15)
  Output : Outport  VectorParamsAs1DForOutWhenUnconnected=off
  wires:
  data lookup/1 -> Output/1
  HDL Counter2/1 -> data lookup/1
  Enable/1 -> HDL Counter2/1

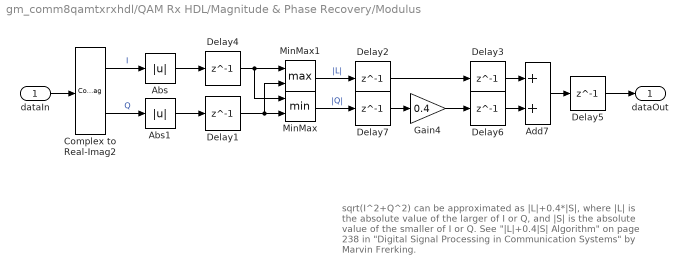
== system gm_comm8qamtxrxhdl/QAM Rx HDL/Magnitude & Phase Recovery/Modulus ==
  note: sqrt(I^2+Q^2) can be approximated as |L|+0.4*|S|,
      | where |L| is the absolute value of the larger of I or Q,
      | and |S| is the absolute value of the smaller of I or Q.
      |
      | See "|L|+0.4|S| Algorithm" on page 238 in "Digital Signal
      | Processing in Communication Systems" by Marvin Frerking.
  dataIn : Inport
  Abs : Abs  SaturateOnIntegerOverflow=off
  Abs1 : Abs  SaturateOnIntegerOverflow=off
  Add7 : Sum
  Complex to Real-Imag2 : ComplexToRealImag
  Delay{1..7} (7 alike) : Delay  DelayLength=1  InitialCondition=0
  Gain4 : Gain  Gain=0.4  OutDataTypeStr=fixdt(1,16,15)
  MinMax : MinMax  Inputs=2
  MinMax1 : MinMax  Function=max  Inputs=2
  dataOut : Outport  VectorParamsAs1DForOutWhenUnconnected=off
  wires:
  Complex to Real-Imag2/1 -> Abs/1  "I"
  Complex to Real-Imag2/2 -> Abs1/1  "Q"
  Delay3/1 -> Add7/1
  Delay5/1 -> dataOut/1
  Delay6/1 -> Add7/2
  Delay4/1 -> MinMax/1, MinMax1/1
  Delay1/1 -> MinMax/2, MinMax1/2
  Delay2/1 -> Delay3/1
  Delay7/1 -> Gain4/1
  Add7/1 -> Delay5/1
  MinMax/1 -> Delay7/1  "|Q|"
  MinMax1/1 -> Delay2/1  "|L|"
  Gain4/1 -> Delay6/1
  Abs/1 -> Delay4/1
  Abs1/1 -> Delay1/1
  dataIn/1 -> Complex to Real-Imag2/1

== system gm_comm8qamtxrxhdl/QAM Rx HDL/Magnitude & Phase Recovery/Preamble Matched Filter ==
  dataIn : Inport
  Add2 : Sum
  Add3 : Sum  Inputs=+-
  Complex to Real-Imag2 : ComplexToRealImag
  Delay{1..4} (4 alike) : Delay  DelayLength=1  InitialCondition=0
  Discrete FIR Filter3 : DiscreteFir  FilterStructure=Direct form transposed  Coefficients=real(fliplr(conj(PreAmb/7)))  CoefDataTypeStr=fixdt(1,16,15)  ProductDataTypeStr=fixdt(1,16,15)  AccumDataTypeStr=fixdt(1,17,15)  OutDataTypeStr=fixdt(1,17,15)
  Discrete FIR Filter4 : DiscreteFir  FilterStructure=Direct form transposed  Coefficients=-real(fliplr(conj(PreAmb/7)))  CoefDataTypeStr=fixdt(1,16,15)  ProductDataTypeStr=fixdt(1,16,15)  AccumDataTypeStr=fixdt(1,17,15)  OutDataTypeStr=fixdt(1,17,15)
  Real-Imag to Complex2 : RealImagToComplex
  dataOut : Outport  VectorParamsAs1DForOutWhenUnconnected=off
  wires:
  dataIn/1 -> Complex to Real-Imag2/1
  Real-Imag to Complex2/1 -> dataOut/1
  Complex to Real-Imag2/2 -> Add3/2, Add2/2
  Complex to Real-Imag2/1 -> Add2/1, Add3/1
  Discrete FIR Filter4/1 -> Delay3/1
  Add2/1 -> Delay4/1
  Discrete FIR Filter3/1 -> Delay2/1
  Add3/1 -> Delay1/1
  Delay4/1 -> Discrete FIR Filter3/1
  Delay2/1 -> Real-Imag to Complex2/1
  Delay3/1 -> Real-Imag to Complex2/2
  Delay1/1 -> Discrete FIR Filter4/1

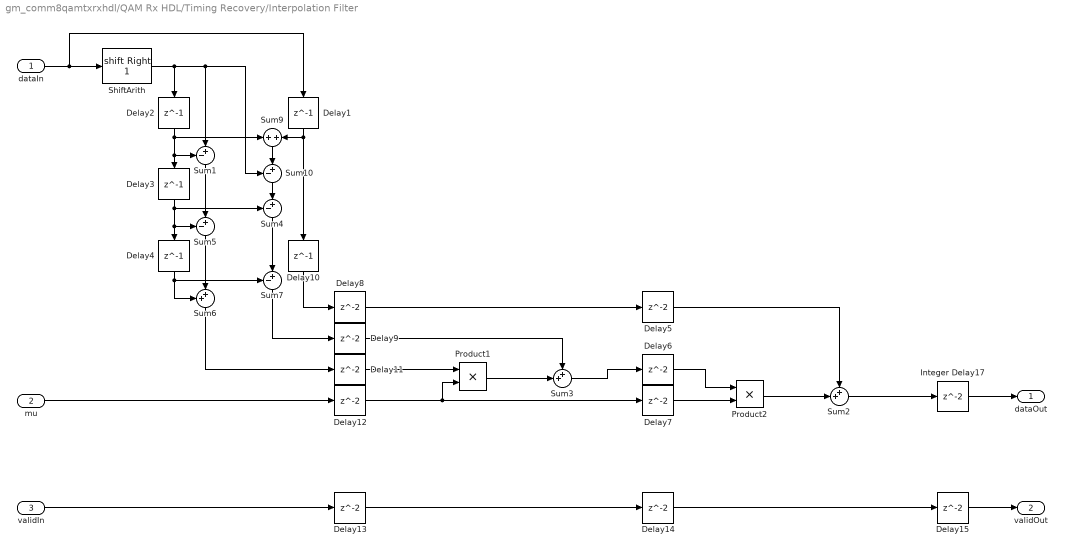
== system gm_comm8qamtxrxhdl/QAM Rx HDL/Timing Recovery/Interpolation Filter  ==
  dataIn : Inport
  mu : Inport  Port=2
  validIn : Inport  Port=3
  Delay{1..4,10} (5 alike) : Delay  DelayLength=1  InitialCondition=0
  Delay{5..9,11..15} (10 alike) : Delay  InitialCondition=0
  Integer Delay17 : Delay  InitialCondition=0
  Product1 : Product  OutDataTypeStr=fixdt(1,16,14)  RndMeth=Zero
  Product2 : Product  OutDataTypeStr=fixdt(1,16,14)  RndMeth=Zero
  ShiftArith : ArithShift  BitShiftNumber=1  BitShiftDirection=Right
  Sum{1,4..5,7,10} (5 alike) : Sum  Inputs=-+|  OutDataTypeStr=fixdt(1,16,14)
  Sum2 : Sum  Inputs=++|  OutDataTypeStr=Inherit: Same as accumulator  AccumDataTypeStr=fixdt(1,16,15)
  Sum3 : Sum  Inputs=++|
  Sum6 : Sum  Inputs=++|  OutDataTypeStr=fixdt(1,16,14)  SaturateOnIntegerOverflow=on
  Sum9 : Sum  Inputs=+|+  OutDataTypeStr=fixdt(1,16,14)
  dataOut : Outport  VectorParamsAs1DForOutWhenUnconnected=off
  validOut : Outport  Port=2  VectorParamsAs1DForOutWhenUnconnected=off
  wires:
  Sum6/1 -> Delay11/1
  Delay15/1 -> validOut/1
  Delay14/1 -> Delay15/1
  Delay13/1 -> Delay14/1
  validIn/1 -> Delay13/1
  Sum9/1 -> Sum10/2
  Sum2/1 -> Integer Delay17/1
  dataIn/1 -> ShiftArith/1, Delay1/1
  Integer Delay17/1 -> dataOut/1
  mu/1 -> Delay12/1
  Sum7/1 -> Delay9/1
  Delay10/1 -> Delay8/1
  Delay5/1 -> Sum2/1
  Delay7/1 -> Product2/2
  Delay12/1 -> Product1/2, Delay7/1
  Delay8/1 -> Delay5/1
  Delay9/1 -> Sum3/1
  Delay11/1 -> Product1/1
  Product1/1 -> Sum3/2
  Product2/1 -> Sum2/2
  Sum3/1 -> Delay6/1
  Delay6/1 -> Product2/1
  Sum4/1 -> Sum7/2
  Sum5/1 -> Sum6/2
  Delay4/1 -> Sum7/1, Sum6/1
  Sum1/1 -> Sum5/2
  Delay3/1 -> Sum4/1, Sum5/1, Delay4/1
  Sum10/1 -> Sum4/2
  Delay2/1 -> Sum1/1, Delay3/1, Sum9/1
  Delay1/1 -> Delay10/1, Sum9/2
  ShiftArith/1 -> Delay2/1, Sum1/2, Sum10/1

== system gm_comm8qamtxrxhdl/QAM Tx HDL/Data Generation & Packetization/Controller FSM ==
  Controller FSM : MATLAB Function  TreatAsAtomicUnit=on  SystemSampleTime=1/qam_params.bitRate
  reset_preamble : Outport  SampleTime=3.33333333333333e-07  VectorParamsAs1DForOutWhenUnconnected=off
  load_preamble : Outport  Port=2  SampleTime=3.33333333333333e-07  VectorParamsAs1DForOutWhenUnconnected=off
  load_data : Outport  Port=3  SampleTime=3.33333333333333e-07  VectorParamsAs1DForOutWhenUnconnected=off
  wires:
  Controller FSM/1(reset_preamble) -> reset_preamble/1
  Controller FSM/3(load_data) -> load_data/1
  Controller FSM/2(load_preamble) -> load_preamble/1
